simulink model "pfb_fft_d3a"  (R2021a)
settings: Solver=VariableStepAuto  StartTime=0.0  StopTime=100.0  RelTol=1e-3
undefined symbols (not defined in the file): i, pfb_coeff_gen_calc
libraries: xbsIndex_r4 x11529, casper_library_misc x39, casper_library_delays x39, xbsReplacements_r4 x2
(part 9 of 118)

== system pfb_fft_d3a/pfb_fir_real/pol1_in8_first_tap ==
  din : Inport
  sync : Inport  Port=2
  coeffs : Inport  Port=3
  Mult : xbsIndex_r4/Mult  precision=Full  arith_type="Signed  (2's comp)"  n_bits=8  bin_pt=2  quantization=Truncate  overflow=Wrap  en=off  latency=mult_latency  use_behavioral_HDL=on  opt=Speed  use_embedded=off  optimum_pipeline=off  pipeline=on  dbl_ovrd=off  use_rpm=on  placement_style=Rectangular shape  block_type=mult
      settings: infoedit=Hardware notes: To use the internal pipeline stage of the dedicated multiplier you must select 'Pipeline for maximum performance'.  xl_area=[0, 0, 0, 0, 0, 0, 0]  block_version=9.1.01
  Reinterpret : xbsIndex_r4/Reinterpret  force_arith_type=on  arith_type="Signed  (2's comp)"  force_bin_pt=on  bin_pt=CoeffBitWidth - 1  block_type=reinterpret
      settings: infoedit="Changes signal type without altering the binary representation.   You can changed the signal between signed and unsigned, and relocate the binary point.<P><P>Hardware notes: In hardware this block costs nothing.<P><P>Example:  Suppose the input is 6 bits wide, signed, with 2 fractional bits, and the output is forced to unsigned with 0 fractional bits.  Then an input of -2.0 (1110.00 in binary 2's complement) becomes an output of 56 (111000 in binary)."  block_version=9.1.01
  Reinterpret2 : xbsIndex_r4/Reinterpret  force_arith_type=on  arith_type="Signed  (2's comp)"  force_bin_pt=on  bin_pt=BitWidthIn - 1  block_type=reinterpret
      settings: infoedit="Changes signal type without altering the binary representation.   You can changed the signal between signed and unsigned, and relocate the binary point.<P><P>Hardware notes: In hardware this block costs nothing.<P><P>Example:  Suppose the input is 6 bits wide, signed, with 2 fractional bits, and the output is forced to unsigned with 0 fractional bits.  Then an input of -2.0 (1110.00 in binary 2's complement) becomes an output of 56 (111000 in binary)."  block_version=9.1.01
  Slice : xbsIndex_r4/Slice  nbits=CoeffBitWidth  boolean_output=off  mode=Lower Bit Location + Width  bit1=0  base1=MSB of Input  bit0=0  base0=LSB of Input  dbl_ovrd=off  block_type=slice
      settings: infoedit="Extracts a given range of bits from each input sample and presents it at the output.  The output type is ordinarily unsigned with binary point at zero, but can be Boolean when the slice is one bit wide.<P><P>Hardware notes: In hardware this block costs nothing."  block_version=9.1.01
  Slice1 : xbsIndex_r4/Slice  nbits=CoeffBitWidth * (TotalTaps - 1)  boolean_output=off  mode=Two Bit Locations  bit1=0  base1=MSB of Input  bit0=CoeffBitWidth  base0=LSB of Input  dbl_ovrd=off  block_type=slice
      settings: infoedit="Extracts a given range of bits from each input sample and presents it at the output.  The output type is ordinarily unsigned with binary point at zero, but can be Boolean when the slice is one bit wide.<P><P>Hardware notes: In hardware this block costs nothing."  block_version=9.1.01
  delay_bram : Subsystem  AncestorBlock=casper_library_delays/delay_bram  mask(delay_bram){DelayLen=2^(PFBSize-n_inputs) * n_pol_blocks, bram_latency=bram_latency, use_dsp48=off, async=off}
      mask prompts: DelayLen "Delay By:"; bram_latency "BRAM Latency"; use_dsp48 "Use DSP48"; async "asynchronous operation"
      mask help: A delay block that uses BRAM for its storage.
      mask init:
      | delay_bram_init(gcb, ...
      |     'DelayLen', DelayLen, ...
      |     'bram_latency', bram_latency, ...
      |     'use_dsp48', use_dsp48, ...
      |     'async', async);
      mask Help: eval('xlWeb(''http://casper.berkeley.edu/wiki/Delay_bram'')')
  sync_delay : casper_library_delays/sync_delay  DelayLen=2^(PFBSize-n_inputs) * n_pol_blocks
      settings: SourceProductName=CASPER DSP Blockset
  dout : Outport  VectorParamsAs1DForOutWhenUnconnected=off
  sync_out : Outport  Port=2  VectorParamsAs1DForOutWhenUnconnected=off
  coeff_out : Outport  Port=3  VectorParamsAs1DForOutWhenUnconnected=off
  taps_out : Outport  Port=4  VectorParamsAs1DForOutWhenUnconnected=off
  wires:
  coeffs/1 -> Slice1/1, Slice/1
  Reinterpret2/1 -> Mult/1
  Reinterpret/1 -> Mult/2
  Slice/1 -> Reinterpret/1
  Slice1/1 -> coeff_out/1
  sync_delay/1 -> sync_out/1
  delay_bram/1(dout) -> dout/1
  Mult/1 -> taps_out/1
  din/1 -> Reinterpret2/1, delay_bram/1(din)
  sync/1 -> sync_delay/1

== system pfb_fft_d3a/pfb_fir_real/pol1_in8_last_tap ==
  din : Inport
  sync : Inport  Port=2
  coeff : Inport  Port=3
  Delay : xbsIndex_r4/Delay  rst=off  infoeditControl=Selection of Reset will increase slice count due to use of real FFs and instead of SRLs  en=off  latency=mult_latency  reg_retiming=off  dbl_ovrd=off  block_type=delay
      settings: xl_area=[0, 0, 0, 0, 0, 0, 0]  block_version=9.1.01
  Mult : xbsIndex_r4/Mult  precision=Full  arith_type="Signed  (2's comp)"  n_bits=8  bin_pt=2  quantization=Truncate  overflow=Wrap  en=off  latency=mult_latency  use_behavioral_HDL=on  opt=Speed  use_embedded=off  optimum_pipeline=off  pipeline=on  dbl_ovrd=off  use_rpm=on  placement_style=Rectangular shape  block_type=mult
      settings: infoedit=Hardware notes: To use the internal pipeline stage of the dedicated multiplier you must select 'Pipeline for maximum performance'.  xl_area=[0, 0, 0, 0, 0, 0, 0]  block_version=9.1.01
  Reinterpret : xbsIndex_r4/Reinterpret  force_arith_type=on  arith_type="Signed  (2's comp)"  force_bin_pt=on  bin_pt=CoeffBitWidth - 1  block_type=reinterpret
      settings: infoedit="Changes signal type without altering the binary representation.   You can changed the signal between signed and unsigned, and relocate the binary point.<P><P>Hardware notes: In hardware this block costs nothing.<P><P>Example:  Suppose the input is 6 bits wide, signed, with 2 fractional bits, and the output is forced to unsigned with 0 fractional bits.  Then an input of -2.0 (1110.00 in binary 2's complement) becomes an output of 56 (111000 in binary)."  block_version=9.1.01
  Reinterpret1 : xbsIndex_r4/Reinterpret  force_arith_type=on  arith_type="Signed  (2's comp)"  force_bin_pt=on  bin_pt=BitWidthIn - 1  block_type=reinterpret
      settings: infoedit="Changes signal type without altering the binary representation.   You can changed the signal between signed and unsigned, and relocate the binary point.<P><P>Hardware notes: In hardware this block costs nothing.<P><P>Example:  Suppose the input is 6 bits wide, signed, with 2 fractional bits, and the output is forced to unsigned with 0 fractional bits.  Then an input of -2.0 (1110.00 in binary 2's complement) becomes an output of 56 (111000 in binary)."  block_version=9.1.01
  tap_out : Outport  VectorParamsAs1DForOutWhenUnconnected=off
  sync_out : Outport  Port=2  VectorParamsAs1DForOutWhenUnconnected=off
  wires:
  Delay/1 -> sync_out/1
  din/1 -> Reinterpret1/1
  sync/1 -> Delay/1
  coeff/1 -> Reinterpret/1
  Reinterpret/1 -> Mult/2
  Mult/1 -> tap_out/1
  Reinterpret1/1 -> Mult/1

== system pfb_fft_d3a/pfb_fir_real/pol1_in8_tap2 ==
  din : Inport
  sync : Inport  Port=2
  coeff : Inport  Port=3
  Mult : xbsIndex_r4/Mult  precision=Full  arith_type="Signed  (2's comp)"  n_bits=8  bin_pt=2  quantization=Truncate  overflow=Wrap  en=off  latency=mult_latency  use_behavioral_HDL=on  opt=Speed  use_embedded=off  optimum_pipeline=off  pipeline=on  dbl_ovrd=off  use_rpm=on  placement_style=Rectangular shape  block_type=mult
      settings: infoedit=Hardware notes: To use the internal pipeline stage of the dedicated multiplier you must select 'Pipeline for maximum performance'.  xl_area=[0, 0, 0, 0, 0, 0, 0]  block_version=9.1.01
  Reinterpret : xbsIndex_r4/Reinterpret  force_arith_type=on  arith_type="Signed  (2's comp)"  force_bin_pt=on  bin_pt=coeff_frac_width  block_type=reinterpret
      settings: infoedit="Changes signal type without altering the binary representation.   You can changed the signal between signed and unsigned, and relocate the binary point.<P><P>Hardware notes: In hardware this block costs nothing.<P><P>Example:  Suppose the input is 6 bits wide, signed, with 2 fractional bits, and the output is forced to unsigned with 0 fractional bits.  Then an input of -2.0 (1110.00 in binary 2's complement) becomes an output of 56 (111000 in binary)."  block_version=9.1.01
  Reinterpret1 : xbsIndex_r4/Reinterpret  force_arith_type=on  arith_type="Signed  (2's comp)"  force_bin_pt=on  bin_pt=data_width - 1  block_type=reinterpret
      settings: infoedit="Changes signal type without altering the binary representation.   You can changed the signal between signed and unsigned, and relocate the binary point.<P><P>Hardware notes: In hardware this block costs nothing.<P><P>Example:  Suppose the input is 6 bits wide, signed, with 2 fractional bits, and the output is forced to unsigned with 0 fractional bits.  Then an input of -2.0 (1110.00 in binary 2's complement) becomes an output of 56 (111000 in binary)."  block_version=9.1.01
  Slice : xbsIndex_r4/Slice  nbits=coeff_width  boolean_output=off  mode=Lower Bit Location + Width  bit1=0  base1=MSB of Input  bit0=0  base0=LSB of Input  dbl_ovrd=off  block_type=slice
      settings: infoedit="Extracts a given range of bits from each input sample and presents it at the output.  The output type is ordinarily unsigned with binary point at zero, but can be Boolean when the slice is one bit wide.<P><P>Hardware notes: In hardware this block costs nothing."  block_version=9.1.01
  Slice1 : xbsIndex_r4/Slice  nbits=0  boolean_output=off  mode=Two Bit Locations  bit1=0  base1=MSB of Input  bit0=coeff_width  base0=LSB of Input  dbl_ovrd=off  block_type=slice
      settings: infoedit="Extracts a given range of bits from each input sample and presents it at the output.  The output type is ordinarily unsigned with binary point at zero, but can be Boolean when the slice is one bit wide.<P><P>Hardware notes: In hardware this block costs nothing."  block_version=9.1.01
  delay_bram : Subsystem  AncestorBlock=casper_library_delays/delay_bram  mask(delay_bram){DelayLen=delay, bram_latency=bram_latency, use_dsp48=off, async=off}
      mask prompts: DelayLen "Delay By:"; bram_latency "BRAM Latency"; use_dsp48 "Use DSP48"; async "asynchronous operation"
      mask help: A delay block that uses BRAM for its storage.
      mask init:
      | delay_bram_init(gcb, ...
      |     'DelayLen', DelayLen, ...
      |     'bram_latency', bram_latency, ...
      |     'use_dsp48', use_dsp48, ...
      |     'async', async);
      mask Help: eval('xlWeb(''http://casper.berkeley.edu/wiki/Delay_bram'')')
  sync_delay : casper_library_delays/sync_delay  DelayLen=delay
      settings: SourceProductName=CASPER DSP Blockset
  dout : Outport  VectorParamsAs1DForOutWhenUnconnected=off
  sync_out : Outport  Port=2  VectorParamsAs1DForOutWhenUnconnected=off
  coeff_out : Outport  Port=3  VectorParamsAs1DForOutWhenUnconnected=off
  taps_out : Outport  Port=4  VectorParamsAs1DForOutWhenUnconnected=off
  wires:
  delay_bram/1(dout) -> dout/1
  din/1 -> Reinterpret1/1, delay_bram/1(din)
  Mult/1 -> taps_out/1
  sync/1 -> sync_delay/1
  sync_delay/1 -> sync_out/1
  coeff/1 -> Slice/1, Slice1/1
  Slice1/1 -> coeff_out/1
  Slice/1 -> Reinterpret/1
  Reinterpret/1 -> Mult/2
  Reinterpret1/1 -> Mult/1

== system pfb_fft_d3a/pfb_fir_real/pol1_in8_tap3 ==
  din : Inport
  sync : Inport  Port=2
  coeff : Inport  Port=3
  Mult : xbsIndex_r4/Mult  precision=Full  arith_type="Signed  (2's comp)"  n_bits=8  bin_pt=2  quantization=Truncate  overflow=Wrap  en=off  latency=mult_latency  use_behavioral_HDL=on  opt=Speed  use_embedded=off  optimum_pipeline=off  pipeline=on  dbl_ovrd=off  use_rpm=on  placement_style=Rectangular shape  block_type=mult
      settings: infoedit=Hardware notes: To use the internal pipeline stage of the dedicated multiplier you must select 'Pipeline for maximum performance'.  xl_area=[0, 0, 0, 0, 0, 0, 0]  block_version=9.1.01
  Reinterpret : xbsIndex_r4/Reinterpret  force_arith_type=on  arith_type="Signed  (2's comp)"  force_bin_pt=on  bin_pt=coeff_frac_width  block_type=reinterpret
      settings: infoedit="Changes signal type without altering the binary representation.   You can changed the signal between signed and unsigned, and relocate the binary point.<P><P>Hardware notes: In hardware this block costs nothing.<P><P>Example:  Suppose the input is 6 bits wide, signed, with 2 fractional bits, and the output is forced to unsigned with 0 fractional bits.  Then an input of -2.0 (1110.00 in binary 2's complement) becomes an output of 56 (111000 in binary)."  block_version=9.1.01
  Reinterpret1 : xbsIndex_r4/Reinterpret  force_arith_type=on  arith_type="Signed  (2's comp)"  force_bin_pt=on  bin_pt=data_width - 1  block_type=reinterpret
      settings: infoedit="Changes signal type without altering the binary representation.   You can changed the signal between signed and unsigned, and relocate the binary point.<P><P>Hardware notes: In hardware this block costs nothing.<P><P>Example:  Suppose the input is 6 bits wide, signed, with 2 fractional bits, and the output is forced to unsigned with 0 fractional bits.  Then an input of -2.0 (1110.00 in binary 2's complement) becomes an output of 56 (111000 in binary)."  block_version=9.1.01
  Slice : xbsIndex_r4/Slice  nbits=coeff_width  boolean_output=off  mode=Lower Bit Location + Width  bit1=0  base1=MSB of Input  bit0=0  base0=LSB of Input  dbl_ovrd=off  block_type=slice
      settings: infoedit="Extracts a given range of bits from each input sample and presents it at the output.  The output type is ordinarily unsigned with binary point at zero, but can be Boolean when the slice is one bit wide.<P><P>Hardware notes: In hardware this block costs nothing."  block_version=9.1.01
  Slice1 : xbsIndex_r4/Slice  nbits=0  boolean_output=off  mode=Two Bit Locations  bit1=0  base1=MSB of Input  bit0=coeff_width  base0=LSB of Input  dbl_ovrd=off  block_type=slice
      settings: infoedit="Extracts a given range of bits from each input sample and presents it at the output.  The output type is ordinarily unsigned with binary point at zero, but can be Boolean when the slice is one bit wide.<P><P>Hardware notes: In hardware this block costs nothing."  block_version=9.1.01
  delay_bram : Subsystem  AncestorBlock=casper_library_delays/delay_bram  mask(delay_bram){DelayLen=delay, bram_latency=bram_latency, use_dsp48=off, async=off}
      mask prompts: DelayLen "Delay By:"; bram_latency "BRAM Latency"; use_dsp48 "Use DSP48"; async "asynchronous operation"
      mask help: A delay block that uses BRAM for its storage.
      mask init:
      | delay_bram_init(gcb, ...
      |     'DelayLen', DelayLen, ...
      |     'bram_latency', bram_latency, ...
      |     'use_dsp48', use_dsp48, ...
      |     'async', async);
      mask Help: eval('xlWeb(''http://casper.berkeley.edu/wiki/Delay_bram'')')
  sync_delay : casper_library_delays/sync_delay  DelayLen=delay
      settings: SourceProductName=CASPER DSP Blockset
  dout : Outport  VectorParamsAs1DForOutWhenUnconnected=off
  sync_out : Outport  Port=2  VectorParamsAs1DForOutWhenUnconnected=off
  coeff_out : Outport  Port=3  VectorParamsAs1DForOutWhenUnconnected=off
  taps_out : Outport  Port=4  VectorParamsAs1DForOutWhenUnconnected=off
  wires:
  delay_bram/1(dout) -> dout/1
  din/1 -> Reinterpret1/1, delay_bram/1(din)
  Mult/1 -> taps_out/1
  sync/1 -> sync_delay/1
  sync_delay/1 -> sync_out/1
  coeff/1 -> Slice/1, Slice1/1
  Slice1/1 -> coeff_out/1
  Slice/1 -> Reinterpret/1
  Reinterpret/1 -> Mult/2
  Reinterpret1/1 -> Mult/1

== system pfb_fft_d3a/fft_wideband_real/fft_biplex_real_4x/bi_real_unscr_4x ==
  sync : Inport
  even : Inport  Port=2
  odd : Inport  Port=3
  c0 : xbsIndex_r4/Constant  const=2^(FFTSize-1)  gui_display_data_type=Fixed-point  arith_type=Unsigned  n_bits=FFTSize  bin_pt=0  preci_type=Single  exp_width=8  frac_width=24  explicit_period=on  period=1  equ=P=C  opselect=C  inp2=PCIN>>17  opr=+  inp1=P  carry=CIN  dbl_ovrd=off  block_type=constant
  c1 : xbsIndex_r4/Constant  const=0  gui_display_data_type=Fixed-point  arith_type=Unsigned  n_bits=FFTSize  bin_pt=0  preci_type=Single  exp_width=8  frac_width=24  explicit_period=on  period=1  equ=P=C  opselect=C  inp2=PCIN>>17  opr=+  inp1=P  carry=CIN  dbl_ovrd=off  block_type=constant
  count : xbsIndex_r4/Counter  cnt_type=Free Running  cnt_to=Inf  operation=Up  start_count=0  cnt_by_val=1  arith_type=Unsigned  n_bits=FFTSize  bin_pt=0  load_pin=off  rst=on  en=off  explicit_period=on  period=1  use_behavioral_HDL=on  implementation=Fabric  dbl_ovrd=off  block_type=counter
  d{0,3..6} (5 alike) : xbsIndex_r4/Delay  rst=off  infoeditControl=Selection of Reset will increase slice count due to use of real FFs and instead of SRLs  en=off  latency=1  reg_retiming=on  dbl_ovrd=off  block_type=delay
  d2 : xbsIndex_r4/Delay  rst=off  infoeditControl=Selection of Reset will increase slice count due to use of real FFs and instead of SRLs  en=off  latency=add_latency + conv_latency + 1  reg_retiming=on  dbl_ovrd=off  block_type=delay
  delay0 : Subsystem  AncestorBlock=casper_library_delays/delay_bram  mask(delay_bram){DelayLen=1024, bram_latency=2, use_dsp48=off, async=off}
      mask prompts: DelayLen "Delay By:"; bram_latency "BRAM Latency"; use_dsp48 "Use DSP48"; async "asynchronous operation"
      mask help: A delay block that uses BRAM for its storage.
      mask init:
      | delay_bram_init(gcb, ...
      |     'DelayLen', DelayLen, ...
      |     'bram_latency', bram_latency, ...
      |     'use_dsp48', use_dsp48, ...
      |     'async', async);
      mask Help: eval('xlWeb(''http://casper.berkeley.edu/wiki/Delay_bram'')')
  delay1 : Subsystem  AncestorBlock=casper_library_delays/delay_bram  mask(delay_bram){DelayLen=1024, bram_latency=2, use_dsp48=off, async=off}
      mask prompts: DelayLen "Delay By:"; bram_latency "BRAM Latency"; use_dsp48 "Use DSP48"; async "asynchronous operation"
      mask help: A delay block that uses BRAM for its storage.
      mask init:
      | delay_bram_init(gcb, ...
      |     'DelayLen', DelayLen, ...
      |     'bram_latency', bram_latency, ...
      |     'use_dsp48', use_dsp48, ...
      |     'async', async);
      mask Help: eval('xlWeb(''http://casper.berkeley.edu/wiki/Delay_bram'')')
  en_even : xbsIndex_r4/Constant  const=1  gui_display_data_type=Fixed-point  arith_type=Boolean  n_bits=1  bin_pt=0  preci_type=Single  exp_width=8  frac_width=24  explicit_period=on  period=1  equ=P=C  opselect=C  inp2=PCIN>>17  opr=+  inp1=P  carry=CIN  dbl_ovrd=off  block_type=constant
  en_odd : xbsIndex_r4/Constant  const=1  gui_display_data_type=Fixed-point  arith_type=Boolean  n_bits=1  bin_pt=0  preci_type=Single  exp_width=8  frac_width=24  explicit_period=on  period=1  equ=P=C  opselect=C  inp2=PCIN>>17  opr=+  inp1=P  carry=CIN  dbl_ovrd=off  block_type=constant
  en_out : xbsIndex_r4/Constant  const=1  gui_display_data_type=Fixed-point  arith_type=Boolean  n_bits=1  bin_pt=0  preci_type=Single  exp_width=8  frac_width=24  explicit_period=on  period=1  equ=P=C  opselect=C  inp2=PCIN>>17  opr=+  inp1=P  carry=CIN  dbl_ovrd=off  block_type=constant
  hilbert0 : Subsystem  AncestorBlock=casper_library_ffts_internal/hilbert  mask(hilbert){n_inputs=2, BitWidth=18, bin_pt_in=17, add_latency=1, conv_latency=conv_latency, misc=off, floating_point=off, float_type=single, exp_width=8, frac_width=24}
      mask prompts: n_inputs "Number simultaneous inputs"; BitWidth "Bit Width"; bin_pt_in "Binary point in"; add_latency "Add Latency"; conv_latency "Convert Latency"; misc "Miscellaneous input"; floating_point "floating point"; float_type "float type"; exp_width "exponent width"; frac_width "fraction width"
      mask help:
      | FFT internal block.
      |
      | Computes (a+b*)/2 and (a-b*)/2i.
      |
      | If a = w + ix and b = y + iz, then:
      | a+b = (w+y)/2 + i(x-z)/2
      | a-b = (x+z)/2 + i(y-w)/2
      mask init:
      | hilbert_init(gcb, ...
      |     'n_inputs', n_inputs, ...
      |     'BitWidth', BitWidth, ...
      |     'bin_pt_in', bin_pt_in, ...
      |     'floating_point', floating_point, ...
      |     'float_type', float_type, ...
      |     'exp_width', exp_width, ...
      |     'frac_width', frac_width, ...    
      |     'add_latency', add_latency, ...
      |     'conv_latency', conv_latency, ...
      |     'misc', misc);
      mask Callback floating_point:
      | onoff = get_param(gcb, 'floating_point');
      | if strcmp(onoff,'on')
      |     enable_fixpt = 'off';
      |     set_param_state(gcb, 'float_type', 'on')
      | 
      |     f_type = get_param(gcb, 'float_type');
      |     if strcmp(f_type,'custom')
      |         set_param_state(gcb, 'exp_width', 'on')
      |         set_param_state(gcb, 'frac_width', 'on')
      |     else
      |         set_param_state(gcb, 'exp_width', 'off')
      |         set_param_state(gcb, 'frac_width', 'off')
      |     end
      | 
      | 
      | else
      |     enable_fixpt = 'on';
      |     set_param_state(gcb, 'float_type', 'off')
      |     set_param_state(gcb, 'exp_width', 'off')
      |     set_param_state(gcb, 'frac_width', 'off')
      | end
      | 
      | set_param_state(gcb, 'BitWidth', enable_fixpt)
      | set_param_state(gcb, 'bin_pt_in', enable_fixpt)
      mask TypeOptions float_type: single | custom
      mask Callback float_type:
      | f_type = get_param(gcb, 'float_type');
      | if strcmp(f_type,'custom')
      |     set_param_state(gcb, 'exp_width', 'on')
      |     set_param_state(gcb, 'frac_width', 'on')
      | else
      |     set_param_state(gcb, 'exp_width', 'off')
      |     set_param_state(gcb, 'frac_width', 'off')
      | end
  hilbert1 : Subsystem  AncestorBlock=casper_library_ffts_internal/hilbert  mask(hilbert){n_inputs=2, BitWidth=18, bin_pt_in=17, add_latency=1, conv_latency=conv_latency, misc=off, floating_point=off, float_type=single, exp_width=8, frac_width=24}
      mask prompts: n_inputs "Number simultaneous inputs"; BitWidth "Bit Width"; bin_pt_in "Binary point in"; add_latency "Add Latency"; conv_latency "Convert Latency"; misc "Miscellaneous input"; floating_point "floating point"; float_type "float type"; exp_width "exponent width"; frac_width "fraction width"
      mask help:
      | FFT internal block.
      |
      | Computes (a+b*)/2 and (a-b*)/2i.
      |
      | If a = w + ix and b = y + iz, then:
      | a+b = (w+y)/2 + i(x-z)/2
      | a-b = (x+z)/2 + i(y-w)/2
      mask init: same as pfb_fft_d3a/fft_wideband_real/fft_biplex_real_4x/bi_real_unscr_4x/hilbert0
      mask Callback floating_point:
      | onoff = get_param(gcb, 'floating_point');
      | if strcmp(onoff,'on')
      |     enable_fixpt = 'off';
      |     set_param_state(gcb, 'float_type', 'on')
      | 
      |     f_type = get_param(gcb, 'float_type');
      |     if strcmp(f_type,'custom')
      |         set_param_state(gcb, 'exp_width', 'on')
      |         set_param_state(gcb, 'frac_width', 'on')
      |     else
      |         set_param_state(gcb, 'exp_width', 'off')
      |         set_param_state(gcb, 'frac_width', 'off')
      |     end
      | 
      | 
      | else
      |     enable_fixpt = 'on';
      |     set_param_state(gcb, 'float_type', 'off')
      |     set_param_state(gcb, 'exp_width', 'off')
      |     set_param_state(gcb, 'frac_width', 'off')
      | end
      | 
      | set_param_state(gcb, 'BitWidth', enable_fixpt)
      | set_param_state(gcb, 'bin_pt_in', enable_fixpt)
      mask TypeOptions float_type: single | custom
      mask Callback float_type:
      | f_type = get_param(gcb, 'float_type');
      | if strcmp(f_type,'custom')
      |     set_param_state(gcb, 'exp_width', 'on')
      |     set_param_state(gcb, 'frac_width', 'on')
      | else
      |     set_param_state(gcb, 'exp_width', 'off')
      |     set_param_state(gcb, 'frac_width', 'off')
      | end
  mirror_spectrum : Subsystem  AncestorBlock=casper_library_ffts_internal/mirror_spectrum  mask(mirror_spectrum){n_inputs=2, FFTSize=11, input_bitwidth=18, bin_pt_in=bin_pt, floating_point=off, float_type=single, exp_width=8, frac_width=24, bram_latency=10, negate_latency=0, negate_mode=logic, async=off}
      mask prompts: n_inputs "Number simultaneous inputs (2*?)"; FFTSize "Size of FFT (2^?)"; input_bitwidth "Input Bit Width"; bin_pt_in "Binary point in"; floating_point "floating point"; float_type "float type"; exp_width "exponent width"; frac_width "fraction width"; bram_latency "BRAM Latency"; negate_latency "Negate Latency"; negate_mode "Negate mode"; async "Asynchronous operation"
      mask help: FFT internal block.
      mask init:
      | mirror_spectrum_init(gcb, ...
      |     'n_inputs', n_inputs, ...
      |     'FFTSize', FFTSize, ...
      |     'input_bitwidth', input_bitwidth, ...
      |     'bin_pt_in', bin_pt_in, ...
      |     'floating_point', floating_point, ...
      |     'float_type', float_type, ...
      |     'exp_width', exp_width, ...
      |     'frac_width', frac_width, ...       
      |     'bram_latency', bram_latency, ...
      |     'negate_latency', negate_latency, ...
      |     'negate_mode', negate_mode, ...
      |     'async', async);
      mask Callback floating_point:
      | onoff = get_param(gcb, 'floating_point');
      | if strcmp(onoff,'on')
      |     enable_fixpt = 'off';
      |     set_param_state(gcb, 'float_type', 'on')
      | 
      |     f_type = get_param(gcb, 'float_type');
      |     if strcmp(f_type,'custom')
      |         set_param_state(gcb, 'exp_width', 'on')
      |         set_param_state(gcb, 'frac_width', 'on')
      |     else
      |         set_param_state(gcb, 'exp_width', 'off')
      |         set_param_state(gcb, 'frac_width', 'off')
      |     end
      | 
      | 
      | else
      |     enable_fixpt = 'on';
      |     set_param_state(gcb, 'float_type', 'off')
      |     set_param_state(gcb, 'exp_width', 'off')
      |     set_param_state(gcb, 'frac_width', 'off')
      | end
      | 
      | set_param_state(gcb, 'input_bitwidth', enable_fixpt)
      | set_param_state(gcb, 'bin_pt_in', enable_fixpt)
      mask TypeOptions float_type: single | custom
      mask Callback float_type:
      | f_type = get_param(gcb, 'float_type');
      | if strcmp(f_type,'custom')
      |     set_param_state(gcb, 'exp_width', 'on')
      |     set_param_state(gcb, 'frac_width', 'on')
      | else
      |     set_param_state(gcb, 'exp_width', 'off')
      |     set_param_state(gcb, 'frac_width', 'off')
      | end
      mask TypeOptions negate_mode: dsp48e | logic
      mask DialogControl ParameterTabVar0 Prompt: Basic
      mask DialogControl ParameterTabVar01 Prompt: Latency
      mask DialogControl ParameterTabVar012 Prompt: Implementation
  mux{0..3} (4 alike) : xbsIndex_r4/Mux  inputs=2  en=off  latency=1  precision=Full  arith_type=Unsigned  n_bits=16  bin_pt=14  quantization=Truncate  overflow=Wrap  dbl_ovrd=off  block_type=mux
  r0 : xbsIndex_r4/Relational  mode=a=b  op_type=Bool  en=off  latency=0  dbl_ovrd=off  block_type=relational
  r1 : xbsIndex_r4/Relational  mode=a=b  op_type=Bool  en=off  latency=0  dbl_ovrd=off  block_type=relational
  reorder_even : Subsystem  AncestorBlock=casper_library_reorder/reorder  mask(reorder){map=[0 512 256 768 128 640 384 896 64 576 320 832 192 704 448 960 32 544 288 800 160 672 416 928 96 608 352 864 224 736 480 992 16 528 272 784 144 656 400 912 80 592 336 848 208 720 464 976 48 560 304 816 176 688 432 944 112 624 368 880 240 752 496 1008 8 520 264 776 136 648 392 904 72 584 328 840 200 712 456 968 40 552 296 808 168 680 424 936 104 616 360 872 232 744 488 1000 24 536 280 792 152 664 408 920 88 600 344 856 216 728 472 984 56 568 312 824 184 696 440 952 120 632 376 888 248 760 504 1016 4 516 260 772 132 644 388 900 68 580 324 836 196 708 452 964 36 548 292 804 164 676 420 932 100 612 356 868 228 740 484 996 20 532 276 788 148 660 404 916 84 596 340 852 212 724 468 980 52 564 308 820 180 692 436 948 116 628 372 884 244 756 500 1012 12 524 268 780 140 652 396 908 76 588 332 844 204 716 460 972 44 556 300 812 172 684 428 940 108 620 364 876 236 748 492 1004 28 540 284 796 156 668 412 924 92 604 348 860 220 732 476 988 60 572 316 828 188 700 444 956 124 636 380 892 252 764 508 1020 2 514 258 770 130 642 386 898 66 578 322 834 194 706 450 962 34 546 290 802 162 674 418 930 98 610 354 866 226 738 482 994 18 530 274 786 146 658 402 914 82 594 338 850 210 722 466 978 50 562 306 818 178 690 434 946 114 626 370 882 242 754 498 1010 10 522 266 778 138 650 394 906 74 586 330 842 202 714 458 970 42 554 298 810 170 682 426 938 106 618 362 874 234 746 490 1002 26 538 282 794 154 666 410 922 90 602 346 858 218 730 474 986 58 570 314 826 186 698 442 954 122 634 378 890 250 762 506 1018 6 518 262 774 134 646 390 902 70 582 326 838 198 710 454 966 38 550 294 806 166 678 422 934 102 614 358 870 230 742 486 998 22 534 278 790 150 662 406 918 86 598 342 854 214 726 470 982 54 566 310 822 182 694 438 950 118 630 374 886 246 758 502 1014 14 526 270 782 142 654 398 910 78 590 334 846 206 718 462 974 46 558 302 814 174 686 430 942 110 622 366 878 238 750 494 1006 30 542 286 798 158 670 414 926 94 606 350 862 222 734 478 990 62 574 318 830 190 702 446 958 126 638 382 894 254 766 510 1022 1 513 257 769 129 641 385 897 65 577 321 833 193 705 449 961 33 545 289 801 161 673 417 929 97 609 353 865 225 737 481 993 17 529 273 785 145 657 401 913 81 593 337 849 209 721 465 977 49 561 305 817 177 689 433 945 113 625 369 881 241 753 497 1009 9 521 265 777 137 649 393 905 73 585 329 841 201 713 457 969 41 553 297 809 169 681 425 937 105 617 361 873 233 745 489 1001 25 537 281 793 153 665 409 921 89 601 345 857 217 729 473 985 57 569 313 825 185 697 441 953 121 633 377 889 249 761 505 1017 5 517 261 773 133 645 389 901 69 581 325 837 197 709 453 965 37 549 293 805 165 677 421 933 101 613 357 869 229 741 485 997 21 533 277 789 149 661 405 917 85 597 341 853 213 725 469 981 53 565 309 821 181 693 437 949 117 629 373 885 245 757 501 1013 13 525 269 781 141 653 397 909 77 589 333 845 205 717 461 973 45 557 301 813 173 685 429 941 109 621 365 877 237 749 493 1005 29 541 285 797 157 669 413 925 93 605 349 861 221 733 477 989 61 573 317 829 189 701 445 957 125 637 381 893 253 765 509 1021 3 515 259 771 131 643 387 899 67 579 323 835 195 707 451 963 35 547 291 803 163 675 419 931 99 611 355 867 227 739 483 995 19 531 275 787 147 659 403 915 83 595 339 851 211 723 467 979 51 563 307 819 179 691 435 947 115 627 371 883 243 755 499 1011 11 523 267 779 139 651 395 907 75 587 331 843 203 715 459 971 43 555 299 811 171 683 427 939 107 619 363 875 235 747 491 1003 27 539 283 795 155 667 411 923 91 603 347 859 219 731 475 987 59 571 315 827 187 699 443 955 123 635 379 891 251 763 507 1019 7 519 263 775 135 647 391 903 71 583 327 839 199 711 455 967 39 551 295 807 167 679 423 935 103 615 359 871 231 743 487 999 23 535 279 791 151 663 407 919 87 599 343 855 215 727 471 983 55 567 311 823 183 695 439 951 119 631 375 887 247 759 503 1015 15 527 271 783 143 655 399 911 79 591 335 847 207 719 463 975 47 559 303 815 175 687 431 943 111 623 367 879 239 751 495 1007 31 543 287 799 159 671 415 927 95 607 351 863 223 735 479 991 63 575 319 831 191 703 447 959 127 639 383 895 255 767 511 1023], n_bits=72, n_inputs=1, bram_latency=2, map_latency=3, fanout_latency=3, double_buffer=0, bram_map=on, software_controlled=off}
      mask prompts: map "Output Order:"; n_bits "Data width in"; n_inputs "Number of inputs"; bram_latency "BRAM Latency"; map_latency "Map Latency"; fanout_latency "Fanout latency"; double_buffer "Double Buffer"; bram_map "Use BlockRAM for Map"; software_controlled "Use runtime software control"
      mask init: same as pfb_fft_d3a/fft_wideband_real/fft_unscrambler/reorder
      settings: AttributesFormatString=order=2
      mask Help: eval('xlWeb(''http://casper.berkeley.edu/wiki/Reorder'')')
  reorder_odd : Subsystem  AncestorBlock=casper_library_reorder/reorder  mask(reorder){map=[1023 511 767 255 895 383 639 127 959 447 703 191 831 319 575 63 991 479 735 223 863 351 607 95 927 415 671 159 799 287 543 31 1007 495 751 239 879 367 623 111 943 431 687 175 815 303 559 47 975 463 719 207 847 335 591 79 911 399 655 143 783 271 527 15 1015 503 759 247 887 375 631 119 951 439 695 183 823 311 567 55 983 471 727 215 855 343 599 87 919 407 663 151 791 279 535 23 999 487 743 231 871 359 615 103 935 423 679 167 807 295 551 39 967 455 711 199 839 327 583 71 903 391 647 135 775 263 519 7 1019 507 763 251 891 379 635 123 955 443 699 187 827 315 571 59 987 475 731 219 859 347 603 91 923 411 667 155 795 283 539 27 1003 491 747 235 875 363 619 107 939 427 683 171 811 299 555 43 971 459 715 203 843 331 587 75 907 395 651 139 779 267 523 11 1011 499 755 243 883 371 627 115 947 435 691 179 819 307 563 51 979 467 723 211 851 339 595 83 915 403 659 147 787 275 531 19 995 483 739 227 867 355 611 99 931 419 675 163 803 291 547 35 963 451 707 195 835 323 579 67 899 387 643 131 771 259 515 3 1021 509 765 253 893 381 637 125 957 445 701 189 829 317 573 61 989 477 733 221 861 349 605 93 925 413 669 157 797 285 541 29 1005 493 749 237 877 365 621 109 941 429 685 173 813 301 557 45 973 461 717 205 845 333 589 77 909 397 653 141 781 269 525 13 1013 501 757 245 885 373 629 117 949 437 693 181 821 309 565 53 981 469 725 213 853 341 597 85 917 405 661 149 789 277 533 21 997 485 741 229 869 357 613 101 933 421 677 165 805 293 549 37 965 453 709 197 837 325 581 69 901 389 645 133 773 261 517 5 1017 505 761 249 889 377 633 121 953 441 697 185 825 313 569 57 985 473 729 217 857 345 601 89 921 409 665 153 793 281 537 25 1001 489 745 233 873 361 617 105 937 425 681 169 809 297 553 41 969 457 713 201 841 329 585 73 905 393 649 137 777 265 521 9 1009 497 753 241 881 369 625 113 945 433 689 177 817 305 561 49 977 465 721 209 849 337 593 81 913 401 657 145 785 273 529 17 993 481 737 225 865 353 609 97 929 417 673 161 801 289 545 33 961 449 705 193 833 321 577 65 897 385 641 129 769 257 513 1 1022 510 766 254 894 382 638 126 958 446 702 190 830 318 574 62 990 478 734 222 862 350 606 94 926 414 670 158 798 286 542 30 1006 494 750 238 878 366 622 110 942 430 686 174 814 302 558 46 974 462 718 206 846 334 590 78 910 398 654 142 782 270 526 14 1014 502 758 246 886 374 630 118 950 438 694 182 822 310 566 54 982 470 726 214 854 342 598 86 918 406 662 150 790 278 534 22 998 486 742 230 870 358 614 102 934 422 678 166 806 294 550 38 966 454 710 198 838 326 582 70 902 390 646 134 774 262 518 6 1018 506 762 250 890 378 634 122 954 442 698 186 826 314 570 58 986 474 730 218 858 346 602 90 922 410 666 154 794 282 538 26 1002 490 746 234 874 362 618 106 938 426 682 170 810 298 554 42 970 458 714 202 842 330 586 74 906 394 650 138 778 266 522 10 1010 498 754 242 882 370 626 114 946 434 690 178 818 306 562 50 978 466 722 210 850 338 594 82 914 402 658 146 786 274 530 18 994 482 738 226 866 354 610 98 930 418 674 162 802 290 546 34 962 450 706 194 834 322 578 66 898 386 642 130 770 258 514 2 1020 508 764 252 892 380 636 124 956 444 700 188 828 316 572 60 988 476 732 220 860 348 604 92 924 412 668 156 796 284 540 28 1004 492 748 236 876 364 620 108 940 428 684 172 812 300 556 44 972 460 716 204 844 332 588 76 908 396 652 140 780 268 524 12 1012 500 756 244 884 372 628 116 948 436 692 180 820 308 564 52 980 468 724 212 852 340 596 84 916 404 660 148 788 276 532 20 996 484 740 228 868 356 612 100 932 420 676 164 804 292 548 36 964 452 708 196 836 324 580 68 900 388 644 132 772 260 516 4 1016 504 760 248 888 376 632 120 952 440 696 184 824 312 568 56 984 472 728 216 856 344 600 88 920 408 664 152 792 280 536 24 1000 488 744 232 872 360 616 104 936 424 680 168 808 296 552 40 968 456 712 200 840 328 584 72 904 392 648 136 776 264 520 8 1008 496 752 240 880 368 624 112 944 432 688 176 816 304 560 48 976 464 720 208 848 336 592 80 912 400 656 144 784 272 528 16 992 480 736 224 864 352 608 96 928 416 672 160 800 288 544 32 960 448 704 192 832 320 576 64 896 384 640 128 768 256 512 0], n_bits=72, n_inputs=1, bram_latency=2, map_latency=3, fanout_latency=3, double_buffer=0, bram_map=on, software_controlled=off}
      mask prompts: map "Output Order:"; n_bits "Data width in"; n_inputs "Number of inputs"; bram_latency "BRAM Latency"; map_latency "Map Latency"; fanout_latency "Fanout latency"; double_buffer "Double Buffer"; bram_map "Use BlockRAM for Map"; software_controlled "Use runtime software control"
      mask init: same as pfb_fft_d3a/fft_wideband_real/fft_unscrambler/reorder
      settings: AttributesFormatString=order=2
      mask Help: eval('xlWeb(''http://casper.berkeley.edu/wiki/Reorder'')')
  reorder_out : Subsystem  AncestorBlock=casper_library_reorder/reorder  mask(reorder){map=[1023 1022 1021 1020 1019 1018 1017 1016 1015 1014 1013 1012 1011 1010 1009 1008 1007 1006 1005 1004 1003 1002 1001 1000 999 998 997 996 995 994 993 992 991 990 989 988 987 986 985 984 983 982 981 980 979 978 977 976 975 974 973 972 971 970 969 968 967 966 965 964 963 962 961 960 959 958 957 956 955 954 953 952 951 950 949 948 947 946 945 944 943 942 941 940 939 938 937 936 935 934 933 932 931 930 929 928 927 926 925 924 923 922 921 920 919 918 917 916 915 914 913 912 911 910 909 908 907 906 905 904 903 902 901 900 899 898 897 896 895 894 893 892 891 890 889 888 887 886 885 884 883 882 881 880 879 878 877 876 875 874 873 872 871 870 869 868 867 866 865 864 863 862 861 860 859 858 857 856 855 854 853 852 851 850 849 848 847 846 845 844 843 842 841 840 839 838 837 836 835 834 833 832 831 830 829 828 827 826 825 824 823 822 821 820 819 818 817 816 815 814 813 812 811 810 809 808 807 806 805 804 803 802 801 800 799 798 797 796 795 794 793 792 791 790 789 788 787 786 785 784 783 782 781 780 779 778 777 776 775 774 773 772 771 770 769 768 767 766 765 764 763 762 761 760 759 758 757 756 755 754 753 752 751 750 749 748 747 746 745 744 743 742 741 740 739 738 737 736 735 734 733 732 731 730 729 728 727 726 725 724 723 722 721 720 719 718 717 716 715 714 713 712 711 710 709 708 707 706 705 704 703 702 701 700 699 698 697 696 695 694 693 692 691 690 689 688 687 686 685 684 683 682 681 680 679 678 677 676 675 674 673 672 671 670 669 668 667 666 665 664 663 662 661 660 659 658 657 656 655 654 653 652 651 650 649 648 647 646 645 644 643 642 641 640 639 638 637 636 635 634 633 632 631 630 629 628 627 626 625 624 623 622 621 620 619 618 617 616 615 614 613 612 611 610 609 608 607 606 605 604 603 602 601 600 599 598 597 596 595 594 593 592 591 590 589 588 587 586 585 584 583 582 581 580 579 578 577 576 575 574 573 572 571 570 569 568 567 566 565 564 563 562 561 560 559 558 557 556 555 554 553 552 551 550 549 548 547 546 545 544 543 542 541 540 539 538 537 536 535 534 533 532 531 530 529 528 527 526 525 524 523 522 521 520 519 518 517 516 515 514 513 512 511 510 509 508 507 506 505 504 503 502 501 500 499 498 497 496 495 494 493 492 491 490 489 488 487 486 485 484 483 482 481 480 479 478 477 476 475 474 473 472 471 470 469 468 467 466 465 464 463 462 461 460 459 458 457 456 455 454 453 452 451 450 449 448 447 446 445 444 443 442 441 440 439 438 437 436 435 434 433 432 431 430 429 428 427 426 425 424 423 422 421 420 419 418 417 416 415 414 413 412 411 410 409 408 407 406 405 404 403 402 401 400 399 398 397 396 395 394 393 392 391 390 389 388 387 386 385 384 383 382 381 380 379 378 377 376 375 374 373 372 371 370 369 368 367 366 365 364 363 362 361 360 359 358 357 356 355 354 353 352 351 350 349 348 347 346 345 344 343 342 341 340 339 338 337 336 335 334 333 332 331 330 329 328 327 326 325 324 323 322 321 320 319 318 317 316 315 314 313 312 311 310 309 308 307 306 305 304 303 302 301 300 299 298 297 296 295 294 293 292 291 290 289 288 287 286 285 284 283 282 281 280 279 278 277 276 275 274 273 272 271 270 269 268 267 266 265 264 263 262 261 260 259 258 257 256 255 254 253 252 251 250 249 248 247 246 245 244 243 242 241 240 239 238 237 236 235 234 233 232 231 230 229 228 227 226 225 224 223 222 221 220 219 218 217 216 215 214 213 212 211 210 209 208 207 206 205 204 203 202 201 200 199 198 197 196 195 194 193 192 191 190 189 188 187 186 185 184 183 182 181 180 179 178 177 176 175 174 173 172 171 170 169 168 167 166 165 164 163 162 161 160 159 158 157 156 155 154 153 152 151 150 149 148 147 146 145 144 143 142 141 140 139 138 137 136 135 134 133 132 131 130 129 128 127 126 125 124 123 122 121 120 119 118 117 116 115 114 113 112 111 110 109 108 107 106 105 104 103 102 101 100 99 98 97 96 95 94 93 92 91 90 89 88 87 86 85 84 83 82 81 80 79 78 77 76 75 74 73 72 71 70 69 68 67 66 65 64 63 62 61 60 59 58 57 56 55 54 53 52 51 50 49 48 47 46 45 44 43 42 41 40 39 38 37 36 35 34 33 32 31 30 29 28 27 26 25 24 23 22 21 20 19 18 17 16 15 14 13 12 11 10 9 8 7 6 5 4 3 2 1 0], n_bits=72, n_inputs=4, bram_latency=bram_latency, map_latency=3, fanout_latency=3, double_buffer=0, bram_map=on, software_controlled=off}
      mask prompts: map "Output Order:"; n_bits "Data width in"; n_inputs "Number of inputs"; bram_latency "BRAM Latency"; map_latency "Map Latency"; fanout_latency "Fanout latency"; double_buffer "Double Buffer"; bram_map "Use BlockRAM for Map"; software_controlled "Use runtime software control"
      mask init: same as pfb_fft_d3a/fft_wideband_real/fft_unscrambler/reorder
      settings: AttributesFormatString=order=2
      mask Help: eval('xlWeb(''http://casper.berkeley.edu/wiki/Reorder'')')
  sync_delay : Subsystem  AncestorBlock=casper_library_delays/sync_delay  mask(sync_delay){DelayLen=1024}
      mask prompts: DelayLen "Delay Length:"
      mask help: Delay an infrequent boolean pulse by the specified number of clocks.
      mask init:
      | BitWidth = max(2, ceil(log2(DelayLen+1)));
      | UseCounter = 1;
      | if DelayLen == 0,
      | 	UseCounter = 0;
      | end
      mask Help: eval('xlWeb(''http://casper.berkeley.edu/wiki/Sync_delay'')')
      mask Display: fprintf('Z^-%d', DelayLen)
  t{0..4} (5 alike) : Terminator
  sync_out : Outport
  pol1_out : Outport  Port=2
  pol2_out : Outport  Port=3
  pol3_out : Outport  Port=4
  pol4_out : Outport  Port=5
  wires:
  even/1 -> reorder_even/3(din0)
  sync/1 -> reorder_even/1(sync), reorder_odd/1(sync)
  odd/1 -> reorder_odd/3(din0)
  reorder_odd/1(sync_out) -> t0/1
  reorder_odd/2(valid) -> t1/1
  reorder_even/2(valid) -> t2/1
  en_even/1 -> reorder_even/2(en)
  en_odd/1 -> reorder_odd/2(en)
  c0/1 -> r0/1
  count/1 -> r0/2, r1/1
  c1/1 -> r1/2
  reorder_odd/3(dout0) -> d0/1
  reorder_even/1(sync_out) -> count/1, d2/1
  r0/1 -> mux0/1, mux3/1
  r1/1 -> mux1/1, mux2/1
  reorder_even/3(dout0) -> mux0/2, mux1/3, mux2/2, mux3/3
  d0/1 -> mux0/3, mux1/2, mux2/3, mux3/2
  d2/1 -> sync_delay/1(In)
  mux0/1 -> hilbert0/1(a)
  mux1/1 -> hilbert0/2(b)
  mux2/1 -> hilbert1/1(a)
  mux3/1 -> hilbert1/2(b)
  hilbert0/1(even) -> delay0/1(din)
  hilbert0/2(odd) -> delay1/1(din)
  delay0/1(dout) -> mirror_spectrum/2(din0), reorder_out/3(din0)
  delay1/1(dout) -> mirror_spectrum/4(din1), reorder_out/4(din1)
  hilbert1/1(even) -> mirror_spectrum/6(din2), reorder_out/5(din2)
  hilbert1/2(odd) -> mirror_spectrum/8(din3), reorder_out/6(din3)
  mirror_spectrum/1(sync_out) -> sync_out/1
  mirror_spectrum/2(dout0) -> pol1_out/1
  mirror_spectrum/3(dout1) -> pol2_out/1
  mirror_spectrum/4(dout2) -> pol3_out/1
  mirror_spectrum/5(dout3) -> pol4_out/1
  sync_delay/1(Out) -> mirror_spectrum/1(sync), reorder_out/1(sync)
  en_out/1 -> reorder_out/2(en)
  reorder_out/1(sync_out) -> t3/1
  reorder_out/2(valid) -> t4/1
  reorder_out/3(dout0) -> d3/1
  d3/1 -> mirror_spectrum/3(reo_in0)
  reorder_out/4(dout1) -> d4/1
  d4/1 -> mirror_spectrum/5(reo_in1)
  reorder_out/5(dout2) -> d5/1
  d5/1 -> mirror_spectrum/7(reo_in2)
  reorder_out/6(dout3) -> d6/1
  d6/1 -> mirror_spectrum/9(reo_in3)
